simulink subsystem "Pitch_Scopes"  (R2025a)
settings: Solver=VariableStepAuto  StartTime=0.0  StopTime=10.0  RelTol=1e-3
Description:
  | Copyright 2025 The MathWorks, Inc.
settings Model: Creator=smiller  LastModifiedBy=smiller

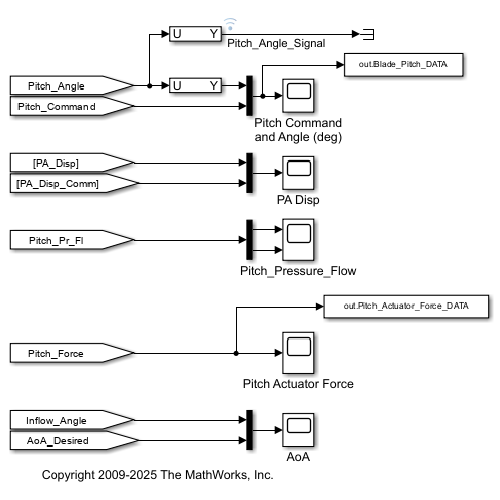
[thumbnail: Simulink's stored preview of the top-level diagram]
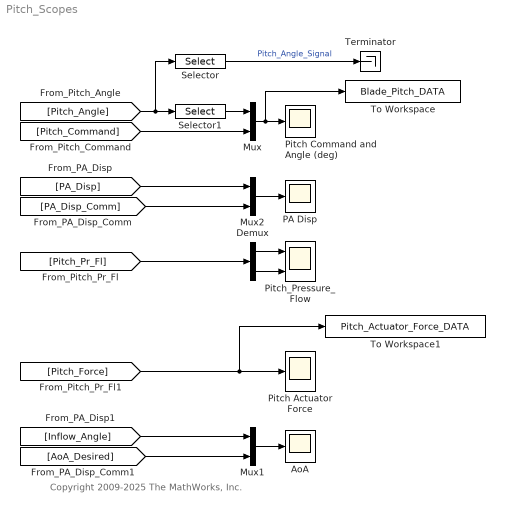
== system Pitch_Scopes ==
  note: Copyright 2009-2025 The MathWorks, Inc.
  AoA : Scope
      settings: TimeSpan=10  ActiveDisplayYMinimum=-1.6  ActiveDisplayYMaximum=-0.9
  Demux : Demux  Outputs=[2 1]
  Mux : Mux  Inputs=2
  Mux1 : Mux  Inputs=2
  Mux2 : Mux  Inputs=2
  PA Disp : Scope
      settings: TimeSpan=10  ActiveDisplayYMinimum=-1.6  ActiveDisplayYMaximum=-0.9  DataLoggingVariableName=ScopeData2
  Pitch Actuator Force : Scope
      settings: TimeSpan=80  ActiveDisplayYMinimum=-78125  ActiveDisplayYMaximum=84375  DataLoggingVariableName=ScopeData3
  Pitch Command and Angle (deg) : Scope
      settings: ActiveDisplayYMinimum=-20  ActiveDisplayYMaximum=80  DataLoggingVariableName=Blade_Pitch_DATA
  Pitch_Pressure_Flow : Scope  NumInputPorts=2
      settings: ActiveDisplayYMinimum=-5  ActiveDisplayYMaximum=20
  Selector : Selector  InputPortWidth=3  IndexOptions=Index vector (dialog)  Indices=[1 ]  OutputSizes=1
  Selector1 : Selector  InputPortWidth=3  IndexOptions=Index vector (dialog)  Indices=[1 ]  OutputSizes=1
  Terminator : Terminator
  To Workspace : ToWorkspace  VariableName=Blade_Pitch_DATA  SaveFormat=Structure With Time  SampleTime=-1
  To Workspace1 : ToWorkspace  VariableName=Pitch_Actuator_Force_DATA  SaveFormat=Structure With Time  SampleTime=-1
  wires:
  [Pitch_Angle] -> Selector/1, Selector1/1
  Selector1/1 -> Mux/1
  Mux1/1 -> AoA/1
  Mux/1 -> To Workspace/1, Pitch Command and Angle (deg)/1
  Selector/1 -> Terminator/1  "Pitch_Angle_Signal"
  Mux2/1 -> PA Disp/1
  [Pitch_Pr_Fl] -> Demux/1
  [PA_Disp_Comm] -> Mux2/2
  Demux/2 -> Pitch_Pressure_Flow/2
  [Pitch_Force] -> To Workspace1/1, Pitch Actuator Force/1
  [Inflow_Angle] -> Mux1/1
  [PA_Disp] -> Mux2/1
  [AoA_Desired] -> Mux1/2
  Demux/1 -> Pitch_Pressure_Flow/1
  [Pitch_Command] -> Mux/2
